simulink model "motion_model"  (Simulink 9.0)
settings: Solver=ode23tb  StartTime=0.0  StopTime=2*pi  MaxStep=0.01  RelTol=1e-3  EnableMultiTasking=on
libraries: aerolibnav x1
settings Model: Creator=me  LastModifiedBy=me
settings DataIOCC: LimitDataPoints=on
settings DebuggingCC: UnderspecifiedInitializationDetection=Simplified  MergeDetectMultiDrivingBlocksExec=error  SolverPrmCheckMsg=warning
settings GRTTargetCC: GeneratePreprocessorConditionals=Disable all
settings ConfigComp: CovSFcnEnable=off

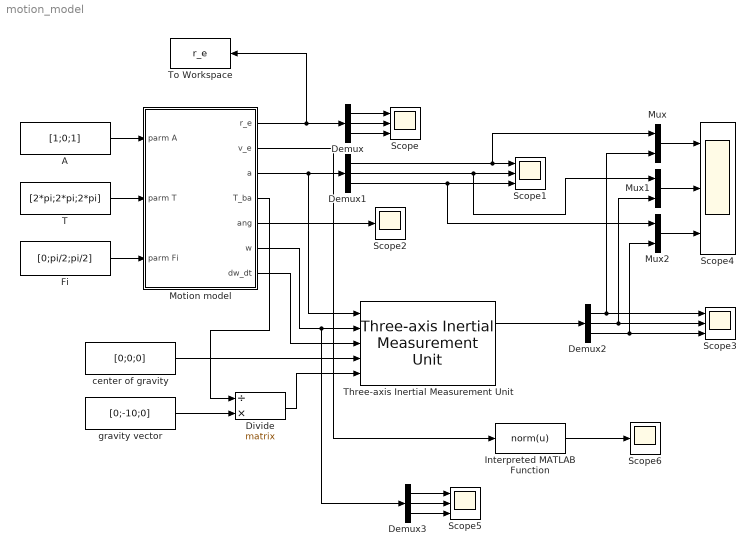
== system motion_model ==
  A : Constant  Value=[1;0;1]
  Demux{,1..3} (4 alike) : Demux  Outputs=3
  Divide : Product  Inputs=/*  Multiplication=Matrix(*)
  Fi : Constant  Value=[0;pi/2;pi/2]
  Interpreted MATLAB Function : MATLABFcn  MATLABFcn=norm(u)
  Motion model : Subsystem
  Mux : Mux  Inputs=2
  Mux1 : Mux  Inputs=2
  Mux2 : Mux  Inputs=2
  Scope{,1,3..5} (5 alike) : Scope  NumInputPorts=3
  Scope2 : Scope
  Scope6 : Scope
  T : Constant  Value=[2*pi;2*pi;2*pi]
  Three-axis Inertial Measurement Unit : aerolibnav/Three-axis Inertial Measurement Unit  units=Metric (MKS)  imu=[0 0 0]  i_Ts=0  dtype_a=on  w_a=190  z_a=0.707  a_sf_cc=[1 0 0; 0 1 0; 0 0 1]  a_bias=[0 0 0]  a_sat="[-inf  -inf  -inf  inf inf inf]"  dtype_g=on  w_g=190  z_g=0.707  g_sf_cc=[1 0 0; 0 1 0; 0 0 1]  g_bias=[0 0 0]  g_sens=[0 0 0]  g_sat="[-inf  -inf  -inf  inf inf inf]"  i_rand=on  i_seeds=[23093 23094 23095 23096 23097 23098]  i_pow=[0.0000 0.0000 0.0000 0.000000 0.000000 0.000000]
  To Workspace : ToWorkspace  VariableName=r_e  SaveFormat=Timeseries  SampleTime=-1
  center of gravity : Constant  Value=[0;0;0]
  gravity vector : Constant  Value=[0;-10;0]
  wires:
  A/1 -> Motion model/1(parm A)
  T/1 -> Motion model/2(parm T)
  Fi/1 -> Motion model/3(parm Fi)
  Demux/3 -> Scope/3
  Demux/1 -> Scope/1
  Demux/2 -> Scope/2
  Motion model/1(r_e) -> To Workspace/1, Demux/1
  Motion model/7(dw_dt) -> Three-axis Inertial Measurement Unit/3
  center of gravity/1 -> Three-axis Inertial Measurement Unit/4
  Demux1/1 -> Mux/1, Scope1/1
  Demux1/2 -> Mux1/1, Scope1/2
  Motion model/3(a) -> Demux1/1, Three-axis Inertial Measurement Unit/1
  Motion model/5(ang) -> Scope2/1
  Demux2/3 -> Mux2/2, Scope3/3
  Demux2/2 -> Mux1/2, Scope3/2
  Three-axis Inertial Measurement Unit/1 -> Demux2/1
  Demux2/1 -> Mux/2, Scope3/1
  Mux/1 -> Scope4/1
  Mux1/1 -> Scope4/2
  Mux2/1 -> Scope4/3
  Demux1/3 -> Mux2/1, Scope1/3
  Demux3/3 -> Scope5/3
  Demux3/1 -> Scope5/1
  Demux3/2 -> Scope5/2
  Motion model/6(w) -> Demux3/1, Three-axis Inertial Measurement Unit/2
  gravity vector/1 -> Divide/2
  Divide/1 -> Three-axis Inertial Measurement Unit/5
  Motion model/4(T_ba) -> Divide/1
  Motion model/2(v_e) -> Interpreted MATLAB Function/1
  Interpreted MATLAB Function/1 -> Scope6/1

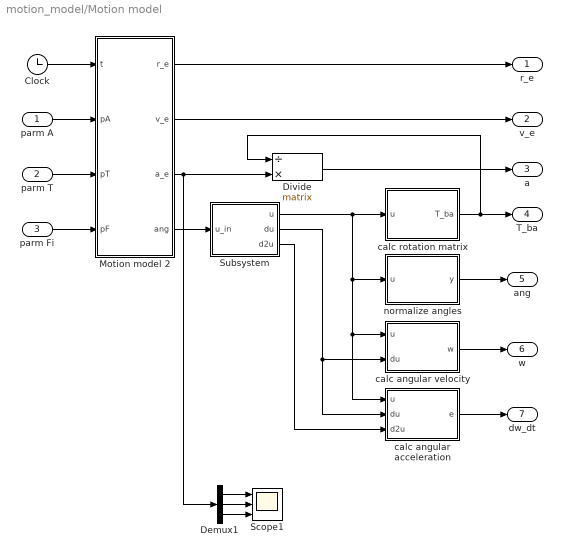
== system motion_model/Motion model ==
  parm A : Inport
  parm T : Inport  Port=2
  parm Fi : Inport  Port=3
  Clock : Clock
  Demux1 : Demux  Outputs=3
  Divide : Product  Inputs=/*  Multiplication=Matrix(*)
  Motion model 2 : MATLAB Function  TreatAsAtomicUnit=on
  Scope1 : Scope  NumInputPorts=3
  Subsystem : Subsystem
  calc angular acceleration : MATLAB Function  TreatAsAtomicUnit=on
  calc angular velocity : MATLAB Function  TreatAsAtomicUnit=on
  calc rotation matrix : MATLAB Function  TreatAsAtomicUnit=on
  normalize angles : MATLAB Function  TreatAsAtomicUnit=on
  r_e : Outport
  v_e : Outport  Port=2
  a : Outport  Port=3
  T_ba : Outport  Port=4
  ang : Outport  Port=5
  w : Outport  Port=6
  dw_dt : Outport  Port=7
  wires:
  parm Fi/1 -> Motion model 2/4(pF)
  parm A/1 -> Motion model 2/2(pA)
  parm T/1 -> Motion model 2/3(pT)
  Subsystem/2(du) -> calc angular acceleration/2(du), calc angular velocity/2(du)
  Subsystem/1(u) -> calc angular acceleration/1(u), calc angular velocity/1(u), normalize angles/1(u), calc rotation matrix/1(u)
  Motion model 2/1(r_e) -> r_e/1
  calc angular acceleration/1(e) -> dw_dt/1
  Subsystem/3(d2u) -> calc angular acceleration/3(d2u)
  calc angular velocity/1(w) -> w/1
  Motion model 2/2(v_e) -> v_e/1
  Clock/1 -> Motion model 2/1(t)
  calc rotation matrix/1(T_ba) -> Divide/1, T_ba/1
  Divide/1 -> a/1
  Demux1/3 -> Scope1/3
  Demux1/2 -> Scope1/2
  Motion model 2/3(a_e) -> Divide/2, Demux1/1
  Demux1/1 -> Scope1/1
  Motion model 2/4(ang) -> Subsystem/1(u_in)
  normalize angles/1(y) -> ang/1

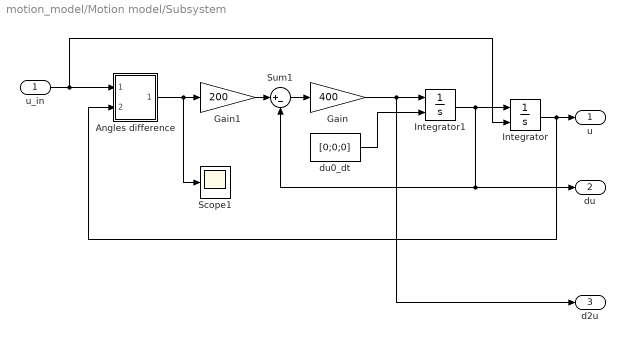
== system motion_model/Motion model/Subsystem ==
  u_in : Inport
  Angles difference : Subsystem
  Gain : Gain  Gain=400
  Gain1 : Gain  Gain=200
  Integrator : Integrator  InitialConditionSource=external
  Integrator1 : Integrator  InitialConditionSource=external
  Scope1 : Scope
  Sum1 : Sum  Inputs=|+-
  du0_dt : Constant  Value=[0;0;0]
  u : Outport
  du : Outport  Port=2
  d2u : Outport  Port=3
  wires:
  Sum1/1 -> Gain/1
  Gain1/1 -> Sum1/1
  Integrator/1 -> Angles difference/2(In2), u/1
  Angles difference/1(Out1) -> Gain1/1, Scope1/1
  Gain/1 -> d2u/1, Integrator1/1
  du0_dt/1 -> Integrator1/2
  Integrator1/1 -> Integrator/1, Sum1/2, du/1
  u_in/1 -> Integrator/2, Angles difference/1(In1)

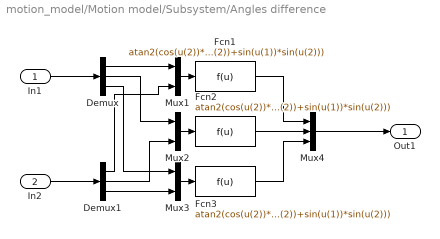
== system motion_model/Motion model/Subsystem/Angles difference ==
  In1 : Inport
  In2 : Inport  Port=2
  Demux : Demux  Outputs=3
  Demux1 : Demux  Outputs=3
  Fcn1 : Fcn  Expr=atan2(cos(u(2))*sin(u(1))-sin(u(2))*cos(u(1)),cos(u(1))*cos(u(2))+sin(u(1))*sin(u(2)))
  Fcn2 : Fcn  Expr=atan2(cos(u(2))*sin(u(1))-sin(u(2))*cos(u(1)),cos(u(1))*cos(u(2))+sin(u(1))*sin(u(2)))
  Fcn3 : Fcn  Expr=atan2(cos(u(2))*sin(u(1))-sin(u(2))*cos(u(1)),cos(u(1))*cos(u(2))+sin(u(1))*sin(u(2)))
  Mux1 : Mux  Inputs=2
  Mux2 : Mux  Inputs=2
  Mux3 : Mux  Inputs=2
  Mux4 : Mux  Inputs=3
  Out1 : Outport
  wires:
  In2/1 -> Demux1/1
  In1/1 -> Demux/1
  Mux2/1 -> Fcn2/1
  Demux/1 -> Mux1/1
  Demux1/2 -> Mux2/2
  Mux4/1 -> Out1/1
  Demux/2 -> Mux2/1
  Fcn1/1 -> Mux4/1
  Fcn2/1 -> Mux4/2
  Demux/3 -> Mux3/1
  Demux1/1 -> Mux1/2
  Demux1/3 -> Mux3/2
  Fcn3/1 -> Mux4/3
  Mux3/1 -> Fcn3/1
  Mux1/1 -> Fcn1/1

== matlab function Motion model/Motion model 2 ==
  data: t input double; r_e output double; pA input double; pT input double; pF input double; v_e output double; a_e output double; ang output double
function [r_e, v_e, a_e, ang] = fcn(t, pA, pT, pF)
%#codegen

    [r_e, v_e, a_e, ~, ang] = f_motion_model2(t, pA, pT, pF);

end

== matlab function Motion model/calc angular velocity ==
  data: u input double; w output double; du input double
function w = fcn(u, du)
%#codegen

w = f_calc_ang_vel(u, du);

== matlab function Motion model/normalize angles ==
  data: u input double; y output double
function y = fcn(u)
%#codegen
y = u;
for i=1:length(y)
    y(i)=f_normalize_angle(u(i));
end

== matlab function Motion model/calc angular acceleration ==
  data: u input double; e output double; du input double; d2u input double
function e = fcn(u, du, d2u)
%#codegen

e = f_calc_ang_accel(u, du, d2u);

== matlab function Motion model/calc rotation matrix ==
  data: u input double; T_ba output double
function T_ba = fcn(u)
%#codegen

T_ba = f_calc_turn_matrix_from_angles(u);
